simulink model "IFOC_BLOCKS"  (R2025a)
settings: Solver=ode4  StartTime=0.0  StopTime=t_stop  FixedStep=h_step  RelTol=1e-3
InitFcn:
  | addpath(fileparts(get_param('IFOC_BLOCKS','FileName'))); bm_drive = 'IFOC'; bm_model = 'IFOC_BLOCKS'; block_model_params;
values from neighbouring files (symbols this model uses):
  Bm = m.B    [block_model_params.m]
  Esw = P.inv.Esw    [block_model_params.m]
  flux_mode_default = c.flux_mode    [block_model_params.m]
  h_step = 5e-6    (= 5e-06)    [block_model_params.m]
  Iref_sw = P.inv.Iref    [block_model_params.m]
  Jm = m.J    [block_model_params.m]
  ke = m.ke    [block_model_params.m]
  kh = m.kh    [block_model_params.m]
  Ki_i = c.Ki_i    [block_model_params.m]
  Ko = c.Ko    [block_model_params.m]
  Kp_i = c.Kp_i    [block_model_params.m]
  Kp_w = c.Kp_w    [block_model_params.m]
  Llr = m.Llr    [block_model_params.m]
  Lls = m.Lls    [block_model_params.m]
  Lm0 = m.Lm0    [block_model_params.m]
  Lm_rated = m.Lm_rated    [block_model_params.m]
  lut_an = P.lut.psi    [block_model_params.m]
  lut_ml = bm_P.lut.psi; end    [block_model_params.m]
  lut_T = P.lut.T(:)'    [block_model_params.m]
  lut_w = P.lut.w(:)'    [block_model_params.m]
  mlp_b1 = double(bm_M.b1(:))    [block_model_params.m]
  mlp_b2 = double(bm_M.b2)    [block_model_params.m]
  mlp_W1 = double(bm_M.W1)    [block_model_params.m]
  mlp_W2 = double(bm_M.W2(:)')    [block_model_params.m]
  mlp_x_mu = double(bm_M.x_mu(:))    [block_model_params.m]
  mlp_x_sd = double(bm_M.x_sd(:))    [block_model_params.m]
  mlp_y_mu = double(bm_M.y_mu)    [block_model_params.m]
  mlp_y_sd = double(bm_M.y_sd)    [block_model_params.m]
  mras_Ki = c.mras_Ki    [block_model_params.m]
  mras_Kp = c.mras_Kp    [block_model_params.m]
  mras_wc = c.mras_wc    [block_model_params.m]
  NT = round(Ts/h)    [block_log_to_thesis.m]    (also in block_model_params.m = round(Ts/h_step))
  pp = m.p    [block_model_params.m]
  psi_k = m.psi_k    [block_model_params.m]
  rad2rpm = 60/(2*pi)    (= 9.54929658551)    [block_model_params.m]
  rce = P.inv.rce    [block_model_params.m]
  rpm2rad = 2*pi/60    (= 0.10471975512)    [block_model_params.m]
  Rr = m.Rr    [block_model_params.m]
  Rs = m.Rs    [block_model_params.m]
  s32 = sqrt(3)/2    [block_model_params.m]
  sat_a = m.sat_a    [block_model_params.m]
  sat_b = m.sat_b    [block_model_params.m]
  sat_on = m.sat_on    [block_model_params.m]
  speed_mode_default = c.speed_mode    [block_model_params.m]
  t_fault = 0.8    [block_model_params.m]
  Te_max = c.Te_max    [block_model_params.m]
  Ts = P.ctrl.Ts    [block_log_to_thesis.m]    (also in block_model_params.m = c.Ts)
  twopi = 2*pi    (= 6.28318530718)    [block_model_params.m]
  Vce0 = P.inv.Vce0    [block_model_params.m]
  Vdc = P.inv.Vdc    [block_model_params.m]
  Vref_sw = P.inv.Vref    [block_model_params.m]
(part 1 of 2)
settings Model: Creator=ironman  LastModifiedBy=ironman
settings DataIOCC: SaveOutput=off  SignalLogging=off  SaveTime=off

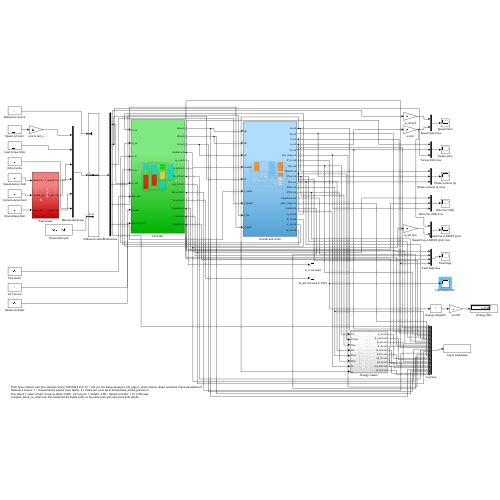
[thumbnail: Simulink's stored preview of the top-level diagram]
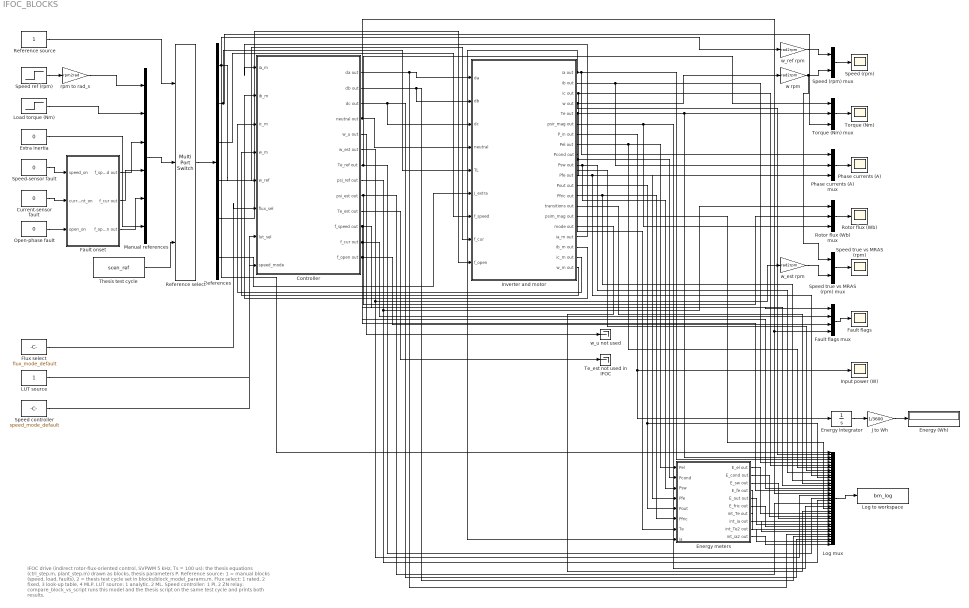
== system IFOC_BLOCKS ==
  note: IFOC drive (indirect rotor-flux-oriented control, SVPWM 5 kHz, Ts = 100 us): the thesis equations (ctrl_step.m, plant_step.m) drawn as blocks, thesis parameters P.
      | Reference source: 1 = manual blocks (speed, load, faults), 2 = thesis test cycle set in blocks/block_model_params.m.
      | Flux select: 1 rated, 2 fixed, 3 look-up table, 4 MLP.  LUT source: 1 analytic, 2 ML.  Speed controller: 1 PI, 2 ZN relay.
      | compare_block_vs_script runs this model and the thesis script on the same test cycle and prints both results.
  Controller : Subsystem
  Current-sensor fault : Constant  Value=0
  Energy (Wh) : Display
  Energy integrator : Integrator
  Energy meters : Subsystem
  Extra inertia : Constant  Value=0
  Fault flags : Scope
      settings: ActiveDisplayYMinimum=-1  ActiveDisplayYMaximum=1
  Fault flags mux : Mux
  Fault onset : Subsystem
  Flux select : Constant  Value=flux_mode_default
  Input power (W) : Scope
      settings: ActiveDisplayYMinimum=-1  ActiveDisplayYMaximum=1
  Inverter and motor : Subsystem
  J to Wh : Gain  Gain=1/3600
  LUT source : Constant
  Load torque (Nm) : Step  Time=0.6  After=13  SampleTime=0
  Log mux : Mux  Inputs=37
  Log to workspace : ToWorkspace  VariableName=bm_log  SaveFormat=Structure With Time  SampleTime=-1
  Manual references : Mux  Inputs=6
  Open-phase fault : Constant  Value=0
  Phase currents (A) : Scope
      settings: ActiveDisplayYMinimum=-1  ActiveDisplayYMaximum=1
  Phase currents (A) mux : Mux  Inputs=3
  Reference select : MultiPortSwitch  Inputs=2  SaturateOnIntegerOverflow=off  InputSameDT=off
  Reference source : Constant
  References : Demux  Outputs=6
  Rotor flux (Wb) : Scope
      settings: ActiveDisplayYMinimum=-1  ActiveDisplayYMaximum=1
  Rotor flux (Wb) mux : Mux  Inputs=3
  Speed (rpm) : Scope
      settings: ActiveDisplayYMinimum=-1  ActiveDisplayYMaximum=1
  Speed (rpm) mux : Mux  Inputs=2
  Speed controller : Constant  Value=speed_mode_default
  Speed ref (rpm) : Step  Time=0.2  After=1000  SampleTime=0
  Speed true vs MRAS (rpm) : Scope
      settings: ActiveDisplayYMinimum=-1  ActiveDisplayYMaximum=1
  Speed true vs MRAS (rpm) mux : Mux  Inputs=2
  Speed-sensor fault : Constant  Value=0
  Te_est not used in IFOC : Terminator
  Thesis test cycle : FromWorkspace  VariableName=scen_ref  SampleTime=Ts  Interpolate=off  OutputAfterFinalValue=Holding final value
  Torque (Nm) : Scope
      settings: ActiveDisplayYMinimum=-1  ActiveDisplayYMaximum=1
  Torque (Nm) mux : Mux  Inputs=3
  rpm to rad_s : Gain  Gain=rpm2rad
  w rpm : Gain  Gain=rad2rpm
  w_est rpm : Gain  Gain=rad2rpm
  w_ref rpm : Gain  Gain=rad2rpm
  w_u not used : Terminator
  wires:
  Speed ref (rpm)/1 -> rpm to rad_s/1
  Speed-sensor fault/1 -> Fault onset/1(speed_on)
  Current-sensor fault/1 -> Fault onset/2(current_on)
  Open-phase fault/1 -> Fault onset/3(open_on)
  rpm to rad_s/1 -> Manual references/1
  Load torque (Nm)/1 -> Manual references/2
  Fault onset/1(f_speed out) -> Manual references/3
  Fault onset/2(f_cur out) -> Manual references/4
  Fault onset/3(f_open out) -> Manual references/5
  Extra inertia/1 -> Manual references/6
  Reference source/1 -> Reference select/1
  Manual references/1 -> Reference select/2
  Thesis test cycle/1 -> Reference select/3
  Reference select/1 -> References/1
  Inverter and motor/17(ia_m out) -> Controller/1(ia_m)
  Inverter and motor/18(ib_m out) -> Controller/2(ib_m)
  Inverter and motor/19(ic_m out) -> Controller/3(ic_m)
  Inverter and motor/20(w_m out) -> Controller/4(w_m)
  References/1 -> Controller/5(w_ref), w_ref rpm/1, Log mux/1
  Flux select/1 -> Controller/6(flux_sel)
  LUT source/1 -> Controller/7(lut_sel)
  Speed controller/1 -> Controller/8(speed_mode)
  Controller/1(da out) -> Inverter and motor/1(da), Log mux/33
  Controller/2(db out) -> Inverter and motor/2(db), Log mux/34
  Controller/3(dc out) -> Inverter and motor/3(dc), Log mux/35
  Controller/4(neutral out) -> Fault flags mux/4, Log mux/17, Inverter and motor/4(neutral)
  References/2 -> Inverter and motor/5(TL), Torque (Nm) mux/3
  References/6 -> Inverter and motor/6(J_extra)
  References/3 -> Inverter and motor/7(f_speed)
  References/4 -> Inverter and motor/8(f_cur)
  References/5 -> Inverter and motor/9(f_open)
  Controller/5(w_u out) -> w_u not used/1
  Controller/10(Te_est out) -> Te_est not used in IFOC/1
  Inverter and motor/4(w out) -> w rpm/1, Log mux/2
  w_ref rpm/1 -> Speed (rpm) mux/1
  w rpm/1 -> Speed (rpm) mux/2, Speed true vs MRAS (rpm) mux/1
  Speed (rpm) mux/1 -> Speed (rpm)/1
  Controller/7(Te_ref out) -> Torque (Nm) mux/1, Log mux/19
  Inverter and motor/5(Te out) -> Torque (Nm) mux/2, Log mux/3, Energy meters/7(Te)
  Torque (Nm) mux/1 -> Torque (Nm)/1
  Controller/8(psi_ref out) -> Rotor flux (Wb) mux/1, Log mux/20
  Controller/9(psi_est out) -> Rotor flux (Wb) mux/2, Log mux/21
  Inverter and motor/6(psir_mag out) -> Rotor flux (Wb) mux/3, Log mux/22
  Rotor flux (Wb) mux/1 -> Rotor flux (Wb)/1
  Inverter and motor/1(ia out) -> Phase currents (A) mux/1, Log mux/4, Energy meters/8(ia)
  Inverter and motor/2(ib out) -> Phase currents (A) mux/2, Log mux/5
  Inverter and motor/3(ic out) -> Phase currents (A) mux/3, Log mux/6
  Phase currents (A) mux/1 -> Phase currents (A)/1
  Controller/6(w_est out) -> w_est rpm/1, Log mux/18
  w_est rpm/1 -> Speed true vs MRAS (rpm) mux/2
  Speed true vs MRAS (rpm) mux/1 -> Speed true vs MRAS (rpm)/1
  Controller/11(f_speed out) -> Fault flags mux/1, Log mux/14
  Controller/12(f_cur out) -> Fault flags mux/2, Log mux/15
  Controller/13(f_open out) -> Fault flags mux/3, Log mux/16
  Fault flags mux/1 -> Fault flags/1
  Inverter and motor/7(P_in out) -> Input power (W)/1, Energy integrator/1
  Energy integrator/1 -> J to Wh/1
  J to Wh/1 -> Energy (Wh)/1
  Inverter and motor/8(Pel out) -> Energy meters/1(Pel), Log mux/7
  Inverter and motor/9(Pcond out) -> Energy meters/2(Pcond), Log mux/8
  Inverter and motor/10(Psw out) -> Energy meters/3(Psw), Log mux/9
  Inverter and motor/11(Pfe out) -> Energy meters/4(Pfe), Log mux/10
  Inverter and motor/12(Pout out) -> Energy meters/5(Pout), Log mux/11
  Inverter and motor/13(Pfric out) -> Energy meters/6(Pfric), Log mux/12
  Inverter and motor/14(transitions out) -> Log mux/13
  Inverter and motor/15(psim_mag out) -> Log mux/23
  Inverter and motor/16(mode out) -> Log mux/24
  Energy meters/1(E_el out) -> Log mux/25
  Energy meters/2(E_cond out) -> Log mux/26
  Energy meters/3(E_sw out) -> Log mux/27
  Energy meters/4(E_fe out) -> Log mux/28
  Energy meters/5(E_out out) -> Log mux/29
  Energy meters/6(E_fric out) -> Log mux/30
  Energy meters/7(int_Te out) -> Log mux/31
  Energy meters/8(int_ia out) -> Log mux/32
  Energy meters/9(int_Te2 out) -> Log mux/36
  Energy meters/10(int_ia2 out) -> Log mux/37
  Log mux/1 -> Log to workspace/1

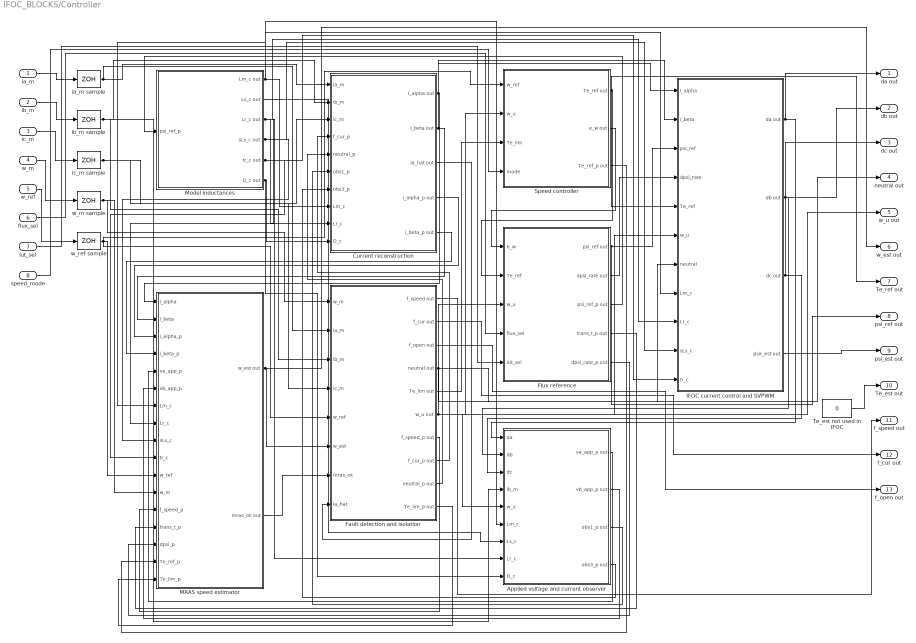
== system IFOC_BLOCKS/Controller ==
  ia_m : Inport
  ib_m : Inport  Port=2
  ic_m : Inport  Port=3
  w_m : Inport  Port=4
  w_ref : Inport  Port=5
  flux_sel : Inport  Port=6
  lut_sel : Inport  Port=7
  speed_mode : Inport  Port=8
  Applied voltage and current observer : Subsystem
  Current reconstruction : Subsystem
  Fault detection and isolation : Subsystem
  Flux reference : Subsystem
  IFOC current control and SVPWM : Subsystem
  MRAS speed estimator : Subsystem
  Model inductances : Subsystem
  Speed controller : Subsystem
  Te_est not used in IFOC : Constant  Value=0
  ia_m sample : ZeroOrderHold  SampleTime=Ts
  ib_m sample : ZeroOrderHold  SampleTime=Ts
  ic_m sample : ZeroOrderHold  SampleTime=Ts
  w_m sample : ZeroOrderHold  SampleTime=Ts
  w_ref sample : ZeroOrderHold  SampleTime=Ts
  da out : Outport
  db out : Outport  Port=2
  dc out : Outport  Port=3
  neutral out : Outport  Port=4
  w_u out : Outport  Port=5
  w_est out : Outport  Port=6
  Te_ref out : Outport  Port=7
  psi_ref out : Outport  Port=8
  psi_est out : Outport  Port=9
  Te_est out : Outport  Port=10
  f_speed out : Outport  Port=11
  f_cur out : Outport  Port=12
  f_open out : Outport  Port=13
  wires:
  ia_m/1 -> ia_m sample/1
  ib_m/1 -> ib_m sample/1
  ic_m/1 -> ic_m sample/1
  w_m/1 -> w_m sample/1
  w_ref/1 -> w_ref sample/1
  Flux reference/3(psi_ref_p out) -> Model inductances/1(psi_ref_p)
  ia_m sample/1 -> Current reconstruction/1(ia_m), Fault detection and isolation/2(ia_m)
  ib_m sample/1 -> Current reconstruction/2(ib_m), Fault detection and isolation/3(ib_m), Applied voltage and current observer/4(ib_m)
  ic_m sample/1 -> Current reconstruction/3(ic_m), Fault detection and isolation/4(ic_m)
  Fault detection and isolation/8(f_cur_p out) -> Current reconstruction/4(f_cur_p)
  Fault detection and isolation/9(neutral_p out) -> Current reconstruction/5(neutral_p)
  Applied voltage and current observer/3(obs1_p out) -> Current reconstruction/6(obs1_p)
  Applied voltage and current observer/4(obs3_p out) -> Current reconstruction/7(obs3_p)
  Model inductances/1(Lm_c out) -> Current reconstruction/8(Lm_c), MRAS speed estimator/7(Lm_c), IFOC current control and SVPWM/8(Lm_c), Applied voltage and current observer/6(Lm_c)
  Model inductances/3(Lr_c out) -> Current reconstruction/9(Lr_c), MRAS speed estimator/8(Lr_c), IFOC current control and SVPWM/9(Lr_c), Applied voltage and current observer/8(Lr_c)
  Model inductances/6(D_c out) -> Current reconstruction/10(D_c), Applied voltage and current observer/9(D_c)
  Current reconstruction/1(i_alpha out) -> MRAS speed estimator/1(i_alpha), IFOC current control and SVPWM/1(i_alpha)
  Current reconstruction/2(i_beta out) -> MRAS speed estimator/2(i_beta), IFOC current control and SVPWM/2(i_beta)
  Current reconstruction/4(i_alpha_p out) -> MRAS speed estimator/3(i_alpha_p)
  Current reconstruction/5(i_beta_p out) -> MRAS speed estimator/4(i_beta_p)
  Applied voltage and current observer/1(va_app_p out) -> MRAS speed estimator/5(va_app_p)
  Applied voltage and current observer/2(vb_app_p out) -> MRAS speed estimator/6(vb_app_p)
  Model inductances/4(sLs_c out) -> MRAS speed estimator/9(sLs_c), IFOC current control and SVPWM/10(sLs_c)
  Model inductances/5(tr_c out) -> MRAS speed estimator/10(tr_c), IFOC current control and SVPWM/11(tr_c)
  w_ref sample/1 -> MRAS speed estimator/11(w_ref), Fault detection and isolation/5(w_ref), Speed controller/1(w_ref)
  w_m sample/1 -> MRAS speed estimator/12(w_m), Fault detection and isolation/1(w_m)
  Fault detection and isolation/7(f_speed_p out) -> MRAS speed estimator/13(f_speed_p)
  Flux reference/4(trans_t_p out) -> MRAS speed estimator/14(trans_t_p)
  Flux reference/5(dpsi_rate_p out) -> MRAS speed estimator/15(dpsi_p)
  Speed controller/3(Te_ref_p out) -> MRAS speed estimator/16(Te_ref_p)
  Fault detection and isolation/10(Te_lim_p out) -> MRAS speed estimator/17(Te_lim_p)
  MRAS speed estimator/1(w_est out) -> Fault detection and isolation/6(w_est), w_est out/1
  MRAS speed estimator/2(mras_ok out) -> Fault detection and isolation/7(mras_ok)
  Current reconstruction/3(ia_hat out) -> Fault detection and isolation/8(ia_hat)
  Fault detection and isolation/6(w_u out) -> Speed controller/2(w_u), Flux reference/3(w_u), IFOC current control and SVPWM/6(w_u), Applied voltage and current observer/5(w_u), w_u out/1
  Fault detection and isolation/5(Te_lim out) -> Speed controller/3(Te_lim)
  speed_mode/1 -> Speed controller/4(mode)
  Speed controller/2(e_w out) -> Flux reference/1(e_w)
  Speed controller/1(Te_ref out) -> Flux reference/2(Te_ref), IFOC current control and SVPWM/5(Te_ref), Te_ref out/1
  flux_sel/1 -> Flux reference/4(flux_sel)
  lut_sel/1 -> Flux reference/5(lut_sel)
  Flux reference/1(psi_ref out) -> IFOC current control and SVPWM/3(psi_ref), psi_ref out/1
  Flux reference/2(dpsi_rate out) -> IFOC current control and SVPWM/4(dpsi_rate)
  Fault detection and isolation/4(neutral out) -> IFOC current control and SVPWM/7(neutral), neutral out/1
  Te_est not used in IFOC/1 -> Te_est out/1
  IFOC current control and SVPWM/1(da out) -> Applied voltage and current observer/1(da), da out/1
  IFOC current control and SVPWM/2(db out) -> Applied voltage and current observer/2(db), db out/1
  IFOC current control and SVPWM/3(dc out) -> Applied voltage and current observer/3(dc), dc out/1
  Model inductances/2(Ls_c out) -> Applied voltage and current observer/7(Ls_c)
  IFOC current control and SVPWM/4(psir_est out) -> psi_est out/1
  Fault detection and isolation/1(f_speed out) -> f_speed out/1
  Fault detection and isolation/2(f_cur out) -> f_cur out/1
  Fault detection and isolation/3(f_open out) -> f_open out/1

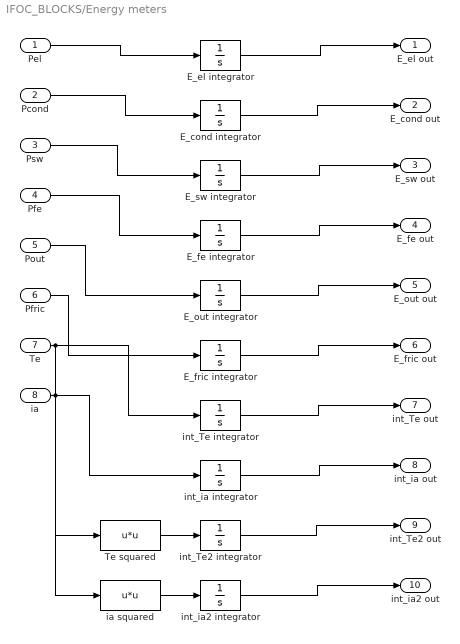
== system IFOC_BLOCKS/Energy meters ==
  Pel : Inport
  Pcond : Inport  Port=2
  Psw : Inport  Port=3
  Pfe : Inport  Port=4
  Pout : Inport  Port=5
  Pfric : Inport  Port=6
  Te : Inport  Port=7
  ia : Inport  Port=8
  E_cond integrator : Integrator
  E_el integrator : Integrator
  E_fe integrator : Integrator
  E_fric integrator : Integrator
  E_out integrator : Integrator
  E_sw integrator : Integrator
  Te squared : Fcn  Expr=u*u
  ia squared : Fcn  Expr=u*u
  int_Te integrator : Integrator
  int_Te2 integrator : Integrator
  int_ia integrator : Integrator
  int_ia2 integrator : Integrator
  E_el out : Outport
  E_cond out : Outport  Port=2
  E_sw out : Outport  Port=3
  E_fe out : Outport  Port=4
  E_out out : Outport  Port=5
  E_fric out : Outport  Port=6
  int_Te out : Outport  Port=7
  int_ia out : Outport  Port=8
  int_Te2 out : Outport  Port=9
  int_ia2 out : Outport  Port=10
  wires:
  Pel/1 -> E_el integrator/1
  E_el integrator/1 -> E_el out/1
  Pcond/1 -> E_cond integrator/1
  E_cond integrator/1 -> E_cond out/1
  Psw/1 -> E_sw integrator/1
  E_sw integrator/1 -> E_sw out/1
  Pfe/1 -> E_fe integrator/1
  E_fe integrator/1 -> E_fe out/1
  Pout/1 -> E_out integrator/1
  E_out integrator/1 -> E_out out/1
  Pfric/1 -> E_fric integrator/1
  E_fric integrator/1 -> E_fric out/1
  Te/1 -> int_Te integrator/1, Te squared/1
  int_Te integrator/1 -> int_Te out/1
  ia/1 -> int_ia integrator/1, ia squared/1
  int_ia integrator/1 -> int_ia out/1
  Te squared/1 -> int_Te2 integrator/1
  int_Te2 integrator/1 -> int_Te2 out/1
  ia squared/1 -> int_ia2 integrator/1
  int_ia2 integrator/1 -> int_ia2 out/1

== system IFOC_BLOCKS/Fault onset ==
  speed_on : Inport
  current_on : Inport  Port=2
  open_on : Inport  Port=3
  Active 1 : Product
  Active 2 : Product
  Active 3 : Product
  Fault time : Step  Time=t_fault  SampleTime=0
  f_speed out : Outport
  f_cur out : Outport  Port=2
  f_open out : Outport  Port=3
  wires:
  speed_on/1 -> Active 1/1
  Fault time/1 -> Active 1/2, Active 2/2, Active 3/2
  Active 1/1 -> f_speed out/1
  current_on/1 -> Active 2/1
  Active 2/1 -> f_cur out/1
  open_on/1 -> Active 3/1
  Active 3/1 -> f_open out/1

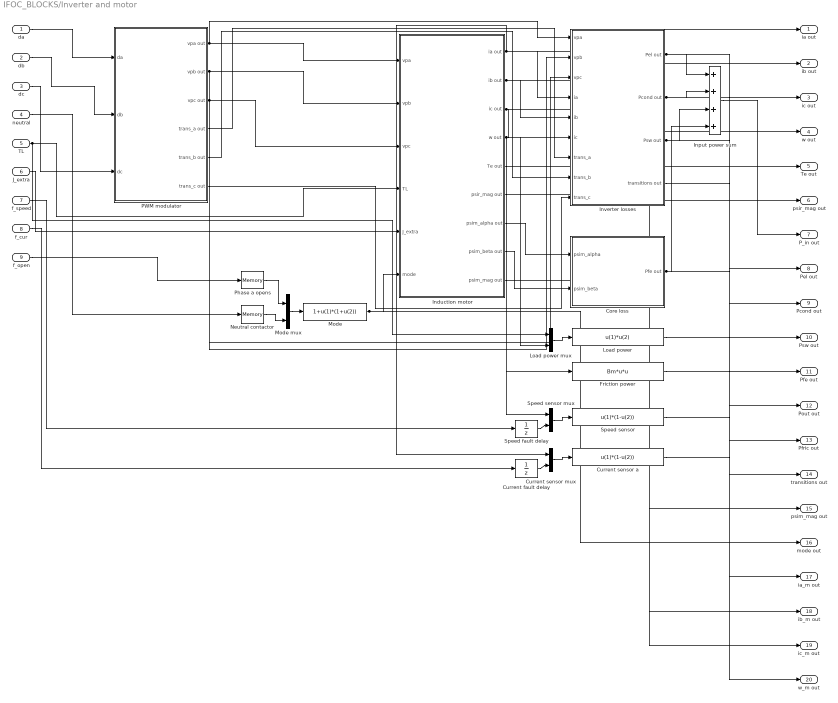
== system IFOC_BLOCKS/Inverter and motor ==
  da : Inport
  db : Inport  Port=2
  dc : Inport  Port=3
  neutral : Inport  Port=4
  TL : Inport  Port=5
  J_extra : Inport  Port=6
  f_speed : Inport  Port=7
  f_cur : Inport  Port=8
  f_open : Inport  Port=9
  Core loss : Subsystem
  Current fault delay : UnitDelay  SampleTime=Ts  HasFrameUpgradeWarning=on
  Current sensor a : Fcn  Expr=u(1)*(1-u(2))
  Current sensor mux : Mux  Inputs=2
  Friction power : Fcn  Expr=Bm*u*u
  Induction motor : Subsystem
  Input power sum : Sum  Inputs=++++
  Inverter losses : Subsystem
  Load power : Fcn  Expr=u(1)*u(2)
  Load power mux : Mux  Inputs=2
  Mode : Fcn  Expr=1+u(1)*(1+u(2))
  Mode mux : Mux  Inputs=2
  Neutral contactor : Memory
  PWM modulator : Subsystem
  Phase a opens : Memory
  Speed fault delay : UnitDelay  SampleTime=Ts  HasFrameUpgradeWarning=on
  Speed sensor : Fcn  Expr=u(1)*(1-u(2))
  Speed sensor mux : Mux  Inputs=2
  ia out : Outport
  ib out : Outport  Port=2
  ic out : Outport  Port=3
  w out : Outport  Port=4
  Te out : Outport  Port=5
  psir_mag out : Outport  Port=6
  P_in out : Outport  Port=7
  Pel out : Outport  Port=8
  Pcond out : Outport  Port=9
  Psw out : Outport  Port=10
  Pfe out : Outport  Port=11
  Pout out : Outport  Port=12
  Pfric out : Outport  Port=13
  transitions out : Outport  Port=14
  psim_mag out : Outport  Port=15
  mode out : Outport  Port=16
  ia_m out : Outport  Port=17
  ib_m out : Outport  Port=18
  ic_m out : Outport  Port=19
  w_m out : Outport  Port=20
  wires:
  neutral/1 -> Neutral contactor/1
  f_open/1 -> Phase a opens/1
  Phase a opens/1 -> Mode mux/1
  Neutral contactor/1 -> Mode mux/2
  Mode mux/1 -> Mode/1
  da/1 -> PWM modulator/1(da)
  db/1 -> PWM modulator/2(db)
  dc/1 -> PWM modulator/3(dc)
  PWM modulator/1(vpa out) -> Induction motor/1(vpa), Inverter losses/1(vpa)
  PWM modulator/2(vpb out) -> Induction motor/2(vpb), Inverter losses/2(vpb)
  PWM modulator/3(vpc out) -> Induction motor/3(vpc), Inverter losses/3(vpc)
  TL/1 -> Induction motor/4(TL), Load power mux/1
  J_extra/1 -> Induction motor/5(J_extra)
  Mode/1 -> Induction motor/6(mode), mode out/1
  Induction motor/1(ia out) -> Inverter losses/4(ia), Current sensor mux/1, ia out/1
  PWM modulator/4(trans_a out) -> Inverter losses/7(trans_a)
  Induction motor/2(ib out) -> Inverter losses/5(ib), ib out/1, ib_m out/1
  PWM modulator/5(trans_b out) -> Inverter losses/8(trans_b)
  Induction motor/3(ic out) -> Inverter losses/6(ic), ic out/1, ic_m out/1
  PWM modulator/6(trans_c out) -> Inverter losses/9(trans_c)
  Induction motor/7(psim_alpha out) -> Core loss/1(psim_alpha)
  Induction motor/8(psim_beta out) -> Core loss/2(psim_beta)
  Induction motor/4(w out) -> Load power mux/2, Friction power/1, Speed sensor mux/1, w out/1
  Load power mux/1 -> Load power/1
  Inverter losses/1(Pel out) -> Input power sum/1, Pel out/1
  Inverter losses/2(Pcond out) -> Input power sum/2, Pcond out/1
  Inverter losses/3(Psw out) -> Input power sum/3, Psw out/1
  Core loss/1(Pfe out) -> Input power sum/4, Pfe out/1
  f_speed/1 -> Speed fault delay/1
  f_cur/1 -> Current fault delay/1
  Speed fault delay/1 -> Speed sensor mux/2
  Speed sensor mux/1 -> Speed sensor/1
  Current fault delay/1 -> Current sensor mux/2
  Current sensor mux/1 -> Current sensor a/1
  Induction motor/5(Te out) -> Te out/1
  Induction motor/6(psir_mag out) -> psir_mag out/1
  Input power sum/1 -> P_in out/1
  Load power/1 -> Pout out/1
  Friction power/1 -> Pfric out/1
  Inverter losses/4(transitions out) -> transitions out/1
  Induction motor/9(psim_mag out) -> psim_mag out/1
  Current sensor a/1 -> ia_m out/1
  Speed sensor/1 -> w_m out/1

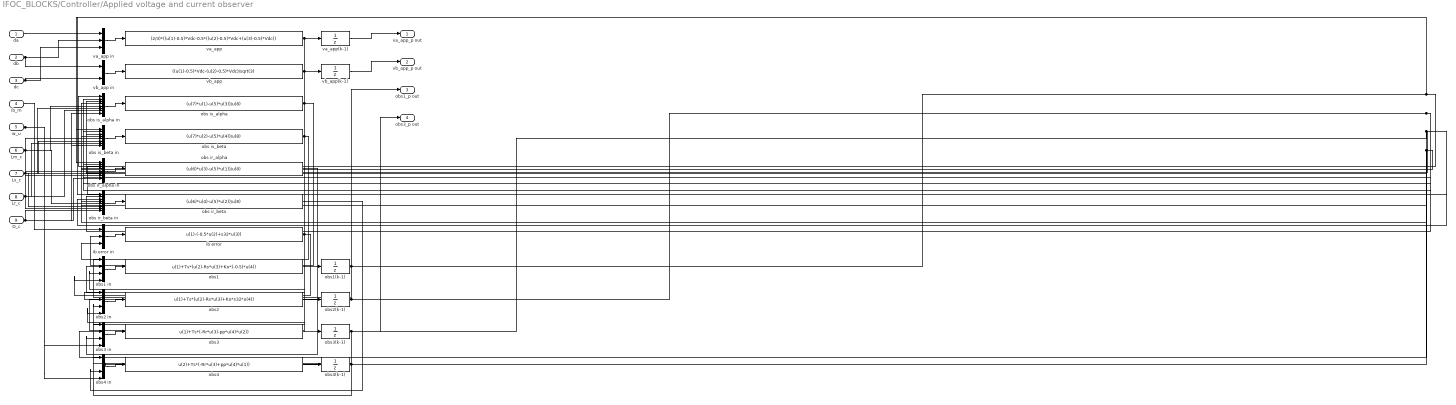
== system IFOC_BLOCKS/Controller/Applied voltage and current observer ==
  da : Inport
  db : Inport  Port=2
  dc : Inport  Port=3
  ib_m : Inport  Port=4
  w_u : Inport  Port=5
  Lm_c : Inport  Port=6
  Ls_c : Inport  Port=7
  Lr_c : Inport  Port=8
  D_c : Inport  Port=9
  ib error : Fcn  Expr=u(1)-(-0.5*u(2)+s32*u(3))
  ib error in : Mux  Inputs=3
  obs ir_alpha : Fcn  Expr=(u(6)*u(3)-u(5)*u(1))/u(8)
  obs ir_alpha in : Mux  Inputs=8
  obs ir_beta : Fcn  Expr=(u(6)*u(4)-u(5)*u(2))/u(8)
  obs ir_beta in : Mux  Inputs=8
  obs is_alpha : Fcn  Expr=(u(7)*u(1)-u(5)*u(3))/u(8)
  obs is_alpha in : Mux  Inputs=8
  obs is_beta : Fcn  Expr=(u(7)*u(2)-u(5)*u(4))/u(8)
  obs is_beta in : Mux  Inputs=8
  obs1 : Fcn  Expr=u(1)+Ts*(u(2)-Rs*u(3)+Ko*(-0.5)*u(4))
  obs1 in : Mux
  obs1(k-1) : UnitDelay  SampleTime=Ts  HasFrameUpgradeWarning=on
  obs2 : Fcn  Expr=u(1)+Ts*(u(2)-Rs*u(3)+Ko*s32*u(4))
  obs2 in : Mux
  obs2(k-1) : UnitDelay  SampleTime=Ts  HasFrameUpgradeWarning=on
  obs3 : Fcn  Expr=u(1)+Ts*(-Rr*u(3)-pp*u(4)*u(2))
  obs3 in : Mux
  obs3(k-1) : UnitDelay  SampleTime=Ts  HasFrameUpgradeWarning=on
  obs4 : Fcn  Expr=u(2)+Ts*(-Rr*u(3)+pp*u(4)*u(1))
  obs4 in : Mux
  obs4(k-1) : UnitDelay  SampleTime=Ts  HasFrameUpgradeWarning=on
  va_app : Fcn  Expr=(2/3)*((u(1)-0.5)*Vdc-0.5*((u(2)-0.5)*Vdc+(u(3)-0.5)*Vdc))
  va_app in : Mux  Inputs=3
  va_app(k-1) : UnitDelay  SampleTime=Ts  HasFrameUpgradeWarning=on
  vb_app : Fcn  Expr=((u(1)-0.5)*Vdc-(u(2)-0.5)*Vdc)/sqrt(3)
  vb_app in : Mux  Inputs=2
  vb_app(k-1) : UnitDelay  SampleTime=Ts  HasFrameUpgradeWarning=on
  va_app_p out : Outport
  vb_app_p out : Outport  Port=2
  obs1_p out : Outport  Port=3
  obs3_p out : Outport  Port=4
  wires:
  da/1 -> va_app in/1
  db/1 -> va_app in/2, vb_app in/1
  dc/1 -> va_app in/3, vb_app in/2
  va_app in/1 -> va_app/1
  va_app/1 -> va_app(k-1)/1, obs1 in/2
  vb_app in/1 -> vb_app/1
  vb_app/1 -> vb_app(k-1)/1, obs2 in/2
  obs1(k-1)/1 -> obs is_alpha in/1, obs is_beta in/1, obs ir_alpha in/1, obs ir_beta in/1, obs1 in/1, obs1_p out/1
  obs2(k-1)/1 -> obs is_alpha in/2, obs is_beta in/2, obs ir_alpha in/2, obs ir_beta in/2, obs2 in/1
  obs3(k-1)/1 -> obs is_alpha in/3, obs is_beta in/3, obs ir_alpha in/3, obs ir_beta in/3, obs3 in/1, obs4 in/1, obs3_p out/1
  obs4(k-1)/1 -> obs is_alpha in/4, obs is_beta in/4, obs ir_alpha in/4, obs ir_beta in/4, obs3 in/2, obs4 in/2
  Lm_c/1 -> obs is_alpha in/5, obs is_beta in/5, obs ir_alpha in/5, obs ir_beta in/5
  Ls_c/1 -> obs is_alpha in/6, obs is_beta in/6, obs ir_alpha in/6, obs ir_beta in/6
  Lr_c/1 -> obs is_alpha in/7, obs is_beta in/7, obs ir_alpha in/7, obs ir_beta in/7
  D_c/1 -> obs is_alpha in/8, obs is_beta in/8, obs ir_alpha in/8, obs ir_beta in/8
  obs is_alpha in/1 -> obs is_alpha/1
  obs is_beta in/1 -> obs is_beta/1
  obs ir_alpha in/1 -> obs ir_alpha/1
  obs ir_beta in/1 -> obs ir_beta/1
  ib_m/1 -> ib error in/1
  obs is_alpha/1 -> ib error in/2, obs1 in/3
  obs is_beta/1 -> ib error in/3, obs2 in/3
  ib error in/1 -> ib error/1
  ib error/1 -> obs1 in/4, obs2 in/4
  obs1 in/1 -> obs1/1
  obs1/1 -> obs1(k-1)/1
  obs2 in/1 -> obs2/1
  obs2/1 -> obs2(k-1)/1
  obs ir_alpha/1 -> obs3 in/3
  w_u/1 -> obs3 in/4, obs4 in/4
  obs3 in/1 -> obs3/1
  obs3/1 -> obs3(k-1)/1
  obs ir_beta/1 -> obs4 in/3
  obs4 in/1 -> obs4/1
  obs4/1 -> obs4(k-1)/1
  va_app(k-1)/1 -> va_app_p out/1
  vb_app(k-1)/1 -> vb_app_p out/1

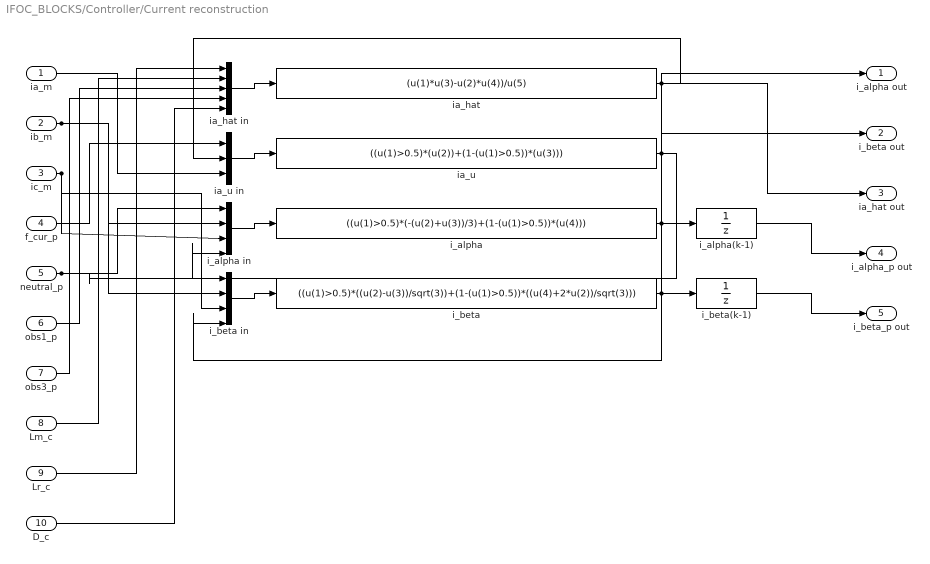
== system IFOC_BLOCKS/Controller/Current reconstruction ==
  ia_m : Inport
  ib_m : Inport  Port=2
  ic_m : Inport  Port=3
  f_cur_p : Inport  Port=4
  neutral_p : Inport  Port=5
  obs1_p : Inport  Port=6
  obs3_p : Inport  Port=7
  Lm_c : Inport  Port=8
  Lr_c : Inport  Port=9
  D_c : Inport  Port=10
  i_alpha : Fcn  Expr=((u(1)>0.5)*(-(u(2)+u(3))/3)+(1-(u(1)>0.5))*(u(4)))
  i_alpha in : Mux
  i_alpha(k-1) : UnitDelay  SampleTime=Ts  HasFrameUpgradeWarning=on
  i_beta : Fcn  Expr=((u(1)>0.5)*((u(2)-u(3))/sqrt(3))+(1-(u(1)>0.5))*((u(4)+2*u(2))/sqrt(3)))
  i_beta in : Mux
  i_beta(k-1) : UnitDelay  SampleTime=Ts  HasFrameUpgradeWarning=on
  ia_hat : Fcn  Expr=(u(1)*u(3)-u(2)*u(4))/u(5)
  ia_hat in : Mux  Inputs=5
  ia_u : Fcn  Expr=((u(1)>0.5)*(u(2))+(1-(u(1)>0.5))*(u(3)))
  ia_u in : Mux  Inputs=3
  i_alpha out : Outport
  i_beta out : Outport  Port=2
  ia_hat out : Outport  Port=3
  i_alpha_p out : Outport  Port=4
  i_beta_p out : Outport  Port=5
  wires:
  Lr_c/1 -> ia_hat in/1
  Lm_c/1 -> ia_hat in/2
  obs1_p/1 -> ia_hat in/3
  obs3_p/1 -> ia_hat in/4
  D_c/1 -> ia_hat in/5
  ia_hat in/1 -> ia_hat/1
  f_cur_p/1 -> ia_u in/1
  ia_hat/1 -> ia_u in/2, ia_hat out/1
  ia_m/1 -> ia_u in/3
  ia_u in/1 -> ia_u/1
  neutral_p/1 -> i_alpha in/1, i_beta in/1
  ib_m/1 -> i_alpha in/2, i_beta in/2
  ic_m/1 -> i_alpha in/3, i_beta in/3
  ia_u/1 -> i_alpha in/4, i_beta in/4
  i_alpha in/1 -> i_alpha/1
  i_alpha/1 -> i_alpha(k-1)/1, i_alpha out/1
  i_beta in/1 -> i_beta/1
  i_beta/1 -> i_beta(k-1)/1, i_beta out/1
  i_alpha(k-1)/1 -> i_alpha_p out/1
  i_beta(k-1)/1 -> i_beta_p out/1

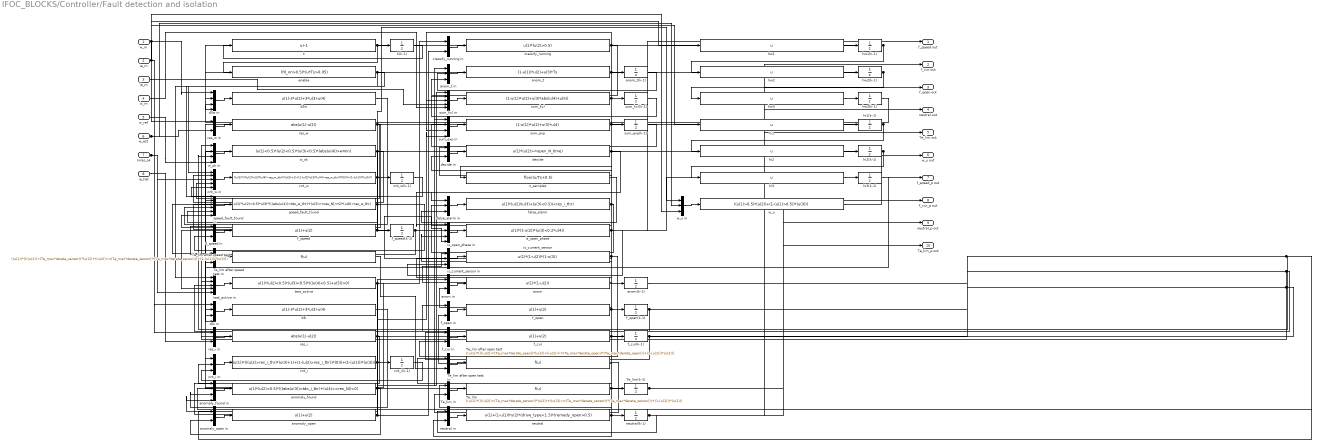
== system IFOC_BLOCKS/Controller/Fault detection and isolation ==
  w_m : Inport
  ia_m : Inport  Port=2
  ib_m : Inport  Port=3
  ic_m : Inport  Port=4
  w_ref : Inport  Port=5
  w_est : Inport  Port=6
  mras_ok : Inport  Port=7
  ia_hat : Inport  Port=8
  Te_lim : Fcn  Expr=((u(1))*((((u(2))<(Te_max*derate_sensor))*(u(2))+((u(2))>=(Te_max*derate_sensor))*(Te_max*derate_sensor)))+(1-(u(1)))*(u(2)))
  Te_lim after open test : Fcn  Expr=((u(1))*((((u(2))<(Te_max*derate_open))*(u(2))+((u(2))>=(Te_max*derate_open))*(Te_max*derate_open)))+(1-(u(1)))*(u(2)))
  Te_lim after open test in : Mux  Inputs=2
  Te_lim after speed test : Fcn  Expr=((u(1))*((((u(2))<(Te_max*derate_sensor))*(u(2))+((u(2))>=(Te_max*derate_sensor))*(Te_max*derate_sensor)))+(1-(u(1)))*(u(2)))
  Te_lim after speed test in : Mux  Inputs=2
  Te_lim in : Mux  Inputs=2
  Te_lim(k-1) : UnitDelay  InitialCondition=Te_max  SampleTime=Ts  HasFrameUpgradeWarning=on
  anom : Fcn  Expr=u(1)*(1-u(2))
  anom in : Mux  Inputs=2
  anom(k-1) : UnitDelay  SampleTime=Ts  HasFrameUpgradeWarning=on
  anom_t : Fcn  Expr=(1-u(1))*u(2)+u(3)*Ts
  anom_t in : Mux  Inputs=3
  anom_t(k-1) : UnitDelay  SampleTime=Ts  HasFrameUpgradeWarning=on
  anomaly_found : Fcn  Expr=u(1)*(u(2)<0.5)*(((abs(u(3))>tdo_i_thr)+(u(4)>=res_N))>0)
  anomaly_found in : Mux
  anomaly_open : Fcn  Expr=u(1)+u(2)
  anomaly_open in : Mux  Inputs=2
  classify_running : Fcn  Expr=u(1)*(u(2)>0.5)
  classify_running in : Mux  Inputs=2
  cnt_i : Fcn  Expr=((u(1))*(((u(2)>res_i_thr)*(u(3)+1)+(1-(u(2)>res_i_thr))*(0)))+(1-(u(1)))*(u(3)))
  cnt_i in : Mux  Inputs=3
  cnt_i(k-1) : UnitDelay  SampleTime=Ts  HasFrameUpgradeWarning=on
  cnt_w : Fcn  Expr=((u(1))*(((u(2)*u(3)*(u(4)>res_w_thr))*(u(5)+1)+(1-(u(2)*u(3)*(u(4)>res_w_thr)))*(0)))+(1-(u(1)))*(u(5)))
  cnt_w in : Mux  Inputs=5
  cnt_w(k-1) : UnitDelay  SampleTime=Ts  HasFrameUpgradeWarning=on
  d3i : Fcn  Expr=u(1)-3*u(2)+3*u(3)-u(4)
  d3i in : Mux
  d3w : Fcn  Expr=u(1)-3*u(2)+3*u(3)-u(4)
  d3w in : Mux
  decide : Fcn  Expr=u(1)*(u(2)>=open_N_time)
  decide in : Mux  Inputs=2
  enable : Fcn  Expr=(fd_on>0.5)*(u*Ts>0.05)
  f_cur : Fcn  Expr=u(1)+u(2)
  f_cur in : Mux  Inputs=2
  f_cur(k-1) : UnitDelay  SampleTime=Ts  HasFrameUpgradeWarning=on
  f_open : Fcn  Expr=u(1)+u(2)
  f_open in : Mux  Inputs=2
  f_open(k-1) : UnitDelay  SampleTime=Ts  HasFrameUpgradeWarning=on
  f_speed : Fcn  Expr=u(1)+u(2)
  f_speed in : Mux  Inputs=2
  f_speed(k-1) : UnitDelay  SampleTime=Ts  HasFrameUpgradeWarning=on
  false_alarm : Fcn  Expr=u(1)*(u(2)/(u(3)+(u(3)<0.5))<res_i_thr)
  false_alarm in : Mux  Inputs=3
  hi1 : Fcn  Expr=u
  hi1(k-1) : UnitDelay  SampleTime=Ts  HasFrameUpgradeWarning=on
  hi2 : Fcn  Expr=u
  hi2(k-1) : UnitDelay  SampleTime=Ts  HasFrameUpgradeWarning=on
  hi3 : Fcn  Expr=u
  hi3(k-1) : UnitDelay  SampleTime=Ts  HasFrameUpgradeWarning=on
  hw1 : Fcn  Expr=u
  hw1(k-1) : UnitDelay  SampleTime=Ts  HasFrameUpgradeWarning=on
  hw2 : Fcn  Expr=u
  hw2(k-1) : UnitDelay  SampleTime=Ts  HasFrameUpgradeWarning=on
  hw3 : Fcn  Expr=u
  hw3(k-1) : UnitDelay  SampleTime=Ts  HasFrameUpgradeWarning=on
  is_current_sensor : Fcn  Expr=u(1)*(1-u(2))*(1-u(3))
  is_current_sensor in : Mux  Inputs=3
  is_open_phase : Fcn  Expr=u(1)*(1-u(2))*(u(3)<0.2*u(4))
  is_open_phase in : Mux
  k : Fcn  Expr=u+1
  k(k-1) : UnitDelay  SampleTime=Ts  HasFrameUpgradeWarning=on
  n_samples : Fcn  Expr=floor(u/Ts+0.5)
  neutral : Fcn  Expr=u(1)+(1-u(1))*u(2)*(drive_type<1.5)*(remedy_open>0.5)
  neutral in : Mux  Inputs=2
  neutral(k-1) : UnitDelay  SampleTime=Ts  HasFrameUpgradeWarning=on
  res_i : Fcn  Expr=abs(u(1)-u(2))
  res_i in : Mux  Inputs=2
  res_w : Fcn  Expr=abs(u(1)-u(2))
  res_w in : Mux  Inputs=2
  speed_fault_found : Fcn  Expr=u(1)*(u(2)<0.5)*u(3)*(((abs(u(4))>tdo_w_thr)+(u(5)>=res_N))>0)*(u(6)>res_w_thr)
  speed_fault_found in : Mux  Inputs=6
  sum_exp : Fcn  Expr=(1-u(1))*u(2)+u(3)*u(4)
  sum_exp in : Mux
  sum_exp(k-1) : UnitDelay  SampleTime=Ts  HasFrameUpgradeWarning=on
  sum_kcl : Fcn  Expr=(1-u(1))*u(2)+u(3)*abs(u(4)+u(5))
  sum_kcl in : Mux  Inputs=5
  sum_kcl(k-1) : UnitDelay  SampleTime=Ts  HasFrameUpgradeWarning=on
  test_active : Fcn  Expr=u(1)*(u(2)<0.5)*(u(3)<0.5)*(((u(4)<0.5)+u(5))>0)
  test_active in : Mux  Inputs=5
  w_ok : Fcn  Expr=(u(1)<0.5)*(u(2)<0.5)*(u(3)<0.5)*(abs(u(4))>wmin)
  w_ok in : Mux
  w_u : Fcn  Expr=((u(1)>0.5)*(u(2))+(1-(u(1)>0.5))*(u(3)))
  w_u in : Mux  Inputs=3
  f_speed out : Outport
  f_cur out : Outport  Port=2
  f_open out : Outport  Port=3
  neutral out : Outport  Port=4
  Te_lim out : Outport  Port=5
  w_u out : Outport  Port=6
  f_speed_p out : Outport  Port=7
  f_cur_p out : Outport  Port=8
  neutral_p out : Outport  Port=9
  Te_lim_p out : Outport  Port=10
  wires:
  k(k-1)/1 -> k/1
  k/1 -> k(k-1)/1, enable/1
  w_m/1 -> d3w in/1, res_w in/1, hw1/1, w_u in/3
  hw1(k-1)/1 -> d3w in/2, hw2/1
  hw2(k-1)/1 -> d3w in/3, hw3/1
  hw3(k-1)/1 -> d3w in/4
  d3w in/1 -> d3w/1
  w_est/1 -> res_w in/2, w_u in/2
  res_w in/1 -> res_w/1
  f_cur(k-1)/1 -> w_ok in/1, test_active in/2, f_cur in/1, f_cur_p out/1
  f_open(k-1)/1 -> w_ok in/2, test_active in/3, f_open in/1
  anom(k-1)/1 -> w_ok in/3, anomaly_found in/2, anomaly_open in/1
  w_ref/1 -> w_ok in/4
  w_ok in/1 -> w_ok/1
  enable/1 -> cnt_w in/1, speed_fault_found in/1, test_active in/1
  w_ok/1 -> cnt_w in/2, speed_fault_found in/3
  mras_ok/1 -> cnt_w in/3, test_active in/5
  res_w/1 -> cnt_w in/4, speed_fault_found in/6
  cnt_w(k-1)/1 -> cnt_w in/5
  cnt_w in/1 -> cnt_w/1
  cnt_w/1 -> cnt_w(k-1)/1, speed_fault_found in/5
  f_speed(k-1)/1 -> speed_fault_found in/2, f_speed in/1, f_speed_p out/1
  d3w/1 -> speed_fault_found in/4
  speed_fault_found in/1 -> speed_fault_found/1
  speed_fault_found/1 -> f_speed in/2, Te_lim after speed test in/1
  f_speed in/1 -> f_speed/1
  f_speed/1 -> f_speed(k-1)/1, test_active in/4, w_u in/1, f_speed out/1
  Te_lim(k-1)/1 -> Te_lim after speed test in/2, Te_lim_p out/1
  Te_lim after speed test in/1 -> Te_lim after speed test/1
  test_active in/1 -> test_active/1
  ia_m/1 -> d3i in/1, res_i in/1, hi1/1
  hi1(k-1)/1 -> d3i in/2, hi2/1
  hi2(k-1)/1 -> d3i in/3, hi3/1
  hi3(k-1)/1 -> d3i in/4
  d3i in/1 -> d3i/1
  ia_hat/1 -> res_i in/2
  res_i in/1 -> res_i/1
  test_active/1 -> cnt_i in/1, anomaly_found in/1, classify_running in/1
  res_i/1 -> cnt_i in/2, sum_exp in/4
  cnt_i(k-1)/1 -> cnt_i in/3
  cnt_i in/1 -> cnt_i/1
  cnt_i/1 -> cnt_i(k-1)/1, anomaly_found in/4
  d3i/1 -> anomaly_found in/3
  anomaly_found in/1 -> anomaly_found/1
  anomaly_found/1 -> anomaly_open in/2, anom_t in/1, sum_kcl in/1, sum_exp in/1
  anomaly_open in/1 -> anomaly_open/1
  anomaly_open/1 -> classify_running in/2, anom in/1
  classify_running in/1 -> classify_running/1
  anom_t(k-1)/1 -> anom_t in/2
  classify_running/1 -> anom_t in/3, sum_kcl in/3, sum_exp in/3, decide in/1
  anom_t in/1 -> anom_t/1
  anom_t/1 -> anom_t(k-1)/1, decide in/2, n_samples/1
  sum_kcl(k-1)/1 -> sum_kcl in/2
  ib_m/1 -> sum_kcl in/4
  ic_m/1 -> sum_kcl in/5
  sum_kcl in/1 -> sum_kcl/1
  sum_kcl/1 -> sum_kcl(k-1)/1, is_open_phase in/3
  sum_exp(k-1)/1 -> sum_exp in/2
  sum_exp in/1 -> sum_exp/1
  sum_exp/1 -> sum_exp(k-1)/1, false_alarm in/2, is_open_phase in/4
  decide in/1 -> decide/1
  decide/1 -> false_alarm in/1, is_open_phase in/1, is_current_sensor in/1, anom in/2
  n_samples/1 -> false_alarm in/3
  false_alarm in/1 -> false_alarm/1
  false_alarm/1 -> is_open_phase in/2, is_current_sensor in/2
  is_open_phase in/1 -> is_open_phase/1
  is_open_phase/1 -> is_current_sensor in/3, f_open in/2, Te_lim after open test in/1, neutral in/2
  is_current_sensor in/1 -> is_current_sensor/1
  anom in/1 -> anom/1
  anom/1 -> anom(k-1)/1
  f_open in/1 -> f_open/1
  f_open/1 -> f_open(k-1)/1, f_open out/1
  is_current_sensor/1 -> f_cur in/2, Te_lim in/1
  f_cur in/1 -> f_cur/1
  f_cur/1 -> f_cur(k-1)/1, f_cur out/1
  Te_lim after speed test/1 -> Te_lim after open test in/2
  Te_lim after open test in/1 -> Te_lim after open test/1
  Te_lim after open test/1 -> Te_lim in/2
  Te_lim in/1 -> Te_lim/1
  Te_lim/1 -> Te_lim(k-1)/1, Te_lim out/1
  neutral(k-1)/1 -> neutral in/1, neutral_p out/1
  neutral in/1 -> neutral/1
  neutral/1 -> neutral(k-1)/1, neutral out/1
  hw1/1 -> hw1(k-1)/1
  hw2/1 -> hw2(k-1)/1
  hw3/1 -> hw3(k-1)/1
  hi1/1 -> hi1(k-1)/1
  hi2/1 -> hi2(k-1)/1
  hi3/1 -> hi3(k-1)/1
  w_u in/1 -> w_u/1
  w_u/1 -> w_u out/1

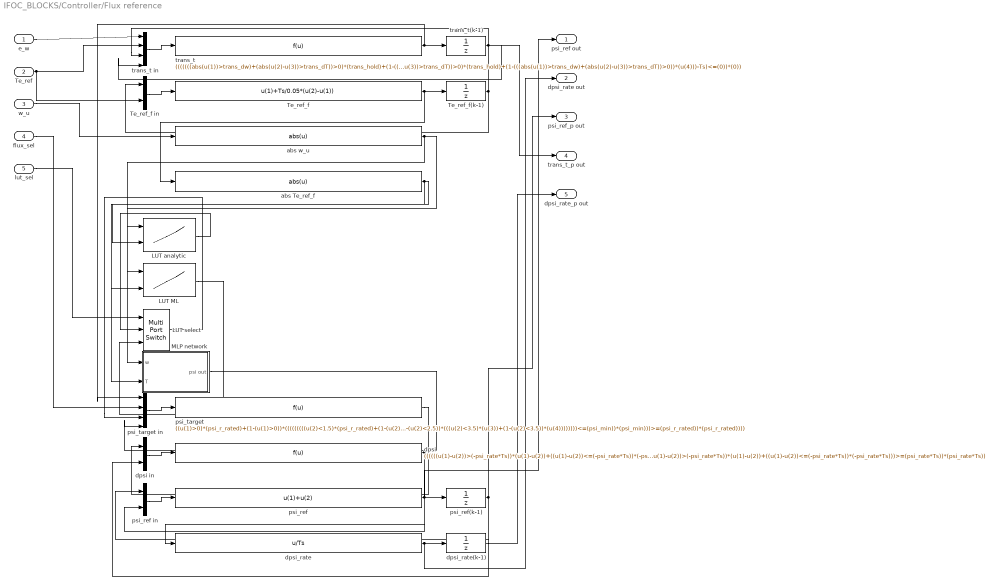
== system IFOC_BLOCKS/Controller/Flux reference ==
  e_w : Inport
  Te_ref : Inport  Port=2
  w_u : Inport  Port=3
  flux_sel : Inport  Port=4
  lut_sel : Inport  Port=5
  LUT ML : Lookup_n-D  BreakpointsForDimension1=lut_w  BreakpointsForDimension2=lut_T  Table=lut_ml  ExtrapMethod=Clip  InternalRulePriority=Speed  RndMeth=Simplest
      settings: InputPortMap=u0,u1
  LUT analytic : Lookup_n-D  BreakpointsForDimension1=lut_w  BreakpointsForDimension2=lut_T  Table=lut_an  ExtrapMethod=Clip  InternalRulePriority=Speed  RndMeth=Simplest
      settings: InputPortMap=u0,u1
  LUT select : MultiPortSwitch  Inputs=2  SaturateOnIntegerOverflow=off  InputSameDT=off
  MLP network : Subsystem
  Te_ref_f : Fcn  Expr=u(1)+Ts/0.05*(u(2)-u(1))
  Te_ref_f in : Mux  Inputs=2
  Te_ref_f(k-1) : UnitDelay  SampleTime=Ts  HasFrameUpgradeWarning=on
  abs Te_ref_f : Fcn  Expr=abs(u)
  abs w_u : Fcn  Expr=abs(u)
  dpsi : Fcn  Expr=((((((u(1)-u(2))>(-psi_rate*Ts))*(u(1)-u(2))+((u(1)-u(2))<=(-psi_rate*Ts))*(-psi_rate*Ts)))<(psi_rate*Ts))*((((u(1)-u(2))>(-psi_rate*Ts))*(u(1)-u(2))+((u(1)-u(2))<=(-psi_rate*Ts))*(-psi_rate*Ts)))+(((((u(1)-u(2))>(-psi_rate*Ts))*(u(1)-u(2))+((u(1)-u(2))<=(-psi_rate*Ts))*(-psi_rate*Ts)))>=(psi_rate*Ts))*(psi_rate*Ts))
  dpsi in : Mux  Inputs=2
  dpsi_rate : Fcn  Expr=u/Ts
  dpsi_rate(k-1) : UnitDelay  SampleTime=Ts  HasFrameUpgradeWarning=on
  psi_ref : Fcn  Expr=u(1)+u(2)
  psi_ref in : Mux  Inputs=2
  psi_ref(k-1) : UnitDelay  SampleTime=Ts  HasFrameUpgradeWarning=on
  psi_target : Fcn  Expr=((u(1)>0)*(psi_r_rated)+(1-(u(1)>0))*(((((((((u(2)<1.5)*(psi_r_rated)+(1-(u(2)<1.5))*(((u(2)<2.5)*(psi_fixed)+(1-(u(2)<2.5))*(((u(2)<3.5)*(u(3))+(1-(u(2)<3.5))*(u(4))))))))>(psi_min))*(((u(2)<1.5)*(psi_r_rated)+(1-(u(2)<1.5))*(((u(2)<2.5)*(psi_fixed)+(1-(u(2)<2.5))*(((u(2)<3.5)*(u(3))+(1-(u(2)<3.5))*(u(4))))))))+((((u(2)<1.5)*(psi_r_rated)+(1-(u(2)<1.5))*(((u(2)<2.5)*(psi_fixed)+(1-(u(2)<2.5))*(((u(2)<3.5)*(u(3))+(1-(u(2)<3.5))*(u(4))))))))<=(psi_min))*(psi_min)))<(psi_r_rated))*((((((u(2)<1.5)*(psi_r_rated)+(1-(u(2)<1.5))*(((u(2)<2.5)*(psi_fixed)+(1-(u(2)<2.5))*(((u(2)<3.5)*(u(3))+(1-(u(2)<3.5))*(u(4))))))))>(psi_min))*(((u(2)<1.5)*(psi_r_rated)+(1-(u(2)<1.5))*(((u(2)<2.5)*(psi_fixed)+(1-(u(2)<2.5))*(((u(2)<3.5)*(u(3))+(1-(u(2)<3.5))*(u(4))))))))+((((u(2)<1.5)*(psi_r_rated)+(1-(u(2)<1.5))*(((u(2)<2.5)*(psi_fixed)+(1-(u(2)<2.5))*(((u(2)<3.5)*(u(3))+(1-(u(2)<3.5))*(u(4))))))))<=(psi_min))*(psi_min)))+(((((((u(2)<1.5)*(psi_r_rated)+(1-(u(2)<1.5))*(((u(2)<2.5)*(psi_fixed)+(1-(u(2)<2.5))*(((u(2)<3.5)*(u(3))+(1-(u(2)<3.5))*(u(4))))))))>(psi_min))*(((u(2)<1.5)*(psi_r_rated)+(1-(u(2)<1.5))*(((u(2)<2.5)*(psi_fixed)+(1-(u(2)<2.5))*(((u(2)<3.5)*(u(3))+(1-(u(2)<3.5))*(u(4))))))))+((((u(2)<1.5)*(psi_r_rated)+(1-(u(2)<1.5))*(((u(2)<2.5)*(psi_fixed)+(1-(u(2)<2.5))*(((u(2)<3.5)*(u(3))+(1-(u(2)<3.5))*(u(4))))))))<=(psi_min))*(psi_min)))>=(psi_r_rated))*(psi_r_rated))))
  psi_target in : Mux
  trans_t : Fcn  Expr=(((((((abs(u(1))>trans_dw)+(abs(u(2)-u(3))>trans_dT))>0)*(trans_hold)+(1-(((abs(u(1))>trans_dw)+(abs(u(2)-u(3))>trans_dT))>0))*(u(4)))-Ts)>(0))*(((((abs(u(1))>trans_dw)+(abs(u(2)-u(3))>trans_dT))>0)*(trans_hold)+(1-(((abs(u(1))>trans_dw)+(abs(u(2)-u(3))>trans_dT))>0))*(u(4)))-Ts)+((((((abs(u(1))>trans_dw)+(abs(u(2)-u(3))>trans_dT))>0)*(trans_hold)+(1-(((abs(u(1))>trans_dw)+(abs(u(2)-u(3))>trans_dT))>0))*(u(4)))-Ts)<=(0))*(0))
  trans_t in : Mux
  trans_t(k-1) : UnitDelay  SampleTime=Ts  HasFrameUpgradeWarning=on
  psi_ref out : Outport
  dpsi_rate out : Outport  Port=2
  psi_ref_p out : Outport  Port=3
  trans_t_p out : Outport  Port=4
  dpsi_rate_p out : Outport  Port=5
  wires:
  e_w/1 -> trans_t in/1
  Te_ref/1 -> trans_t in/2, Te_ref_f in/2
  Te_ref_f(k-1)/1 -> trans_t in/3, Te_ref_f in/1
  trans_t(k-1)/1 -> trans_t in/4, trans_t_p out/1
  trans_t in/1 -> trans_t/1
  trans_t/1 -> trans_t(k-1)/1, psi_target in/1
  Te_ref_f in/1 -> Te_ref_f/1
  Te_ref_f/1 -> Te_ref_f(k-1)/1, abs Te_ref_f/1
  w_u/1 -> abs w_u/1
  abs w_u/1 -> LUT analytic/1, LUT ML/1, MLP network/1(w)
  abs Te_ref_f/1 -> LUT analytic/2, LUT ML/2, MLP network/2(T)
  lut_sel/1 -> LUT select/1
  LUT analytic/1 -> LUT select/2
  LUT ML/1 -> LUT select/3
  flux_sel/1 -> psi_target in/2
  LUT select/1 -> psi_target in/3
  MLP network/1(psi out) -> psi_target in/4
  psi_target in/1 -> psi_target/1
  psi_target/1 -> dpsi in/1
  psi_ref(k-1)/1 -> dpsi in/2, psi_ref in/1, psi_ref_p out/1
  dpsi in/1 -> dpsi/1
  dpsi/1 -> psi_ref in/2, dpsi_rate/1
  psi_ref in/1 -> psi_ref/1
  psi_ref/1 -> psi_ref(k-1)/1, psi_ref out/1
  dpsi_rate/1 -> dpsi_rate(k-1)/1, dpsi_rate out/1
  dpsi_rate(k-1)/1 -> dpsi_rate_p out/1

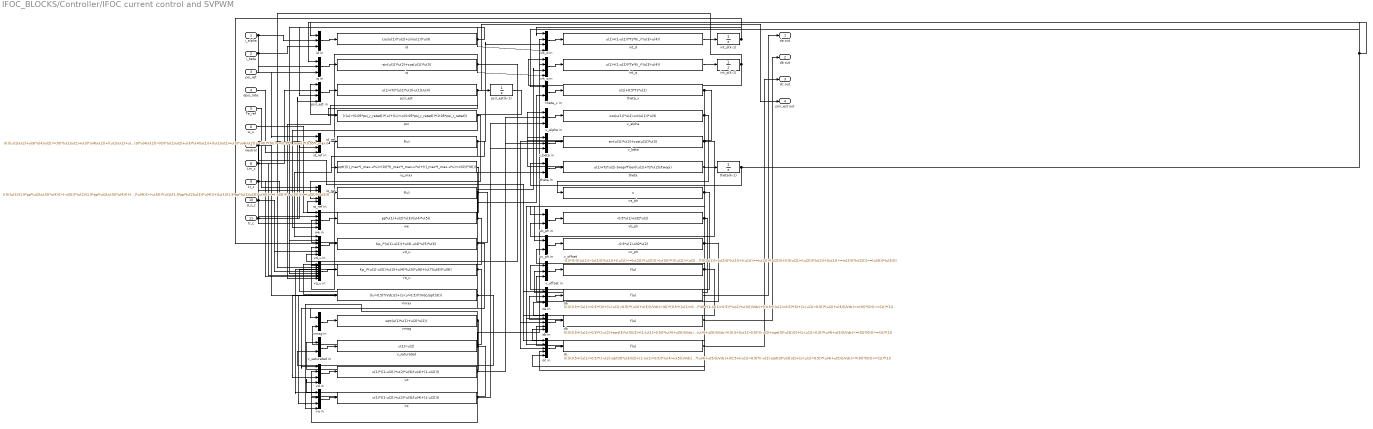
== system IFOC_BLOCKS/Controller/IFOC current control and SVPWM ==
  i_alpha : Inport
  i_beta : Inport  Port=2
  psi_ref : Inport  Port=3
  dpsi_rate : Inport  Port=4
  Te_ref : Inport  Port=5
  w_u : Inport  Port=6
  neutral : Inport  Port=7
  Lm_c : Inport  Port=8
  Lr_c : Inport  Port=9
  sLs_c : Inport  Port=10
  tr_c : Inport  Port=11
  Vmax : Fcn  Expr=((u>0.5)*(Vdc/2)+(1-(u>0.5))*(Vdc/sqrt(3)))
  da : Fcn  Expr=((((((0.5+((u(1)>0.5)*(0)+(1-(u(1)>0.5))*(u(2)+u(3)))/Vdc)>(0))*(0.5+((u(1)>0.5)*(0)+(1-(u(1)>0.5))*(u(2)+u(3)))/Vdc)+((0.5+((u(1)>0.5)*(0)+(1-(u(1)>0.5))*(u(2)+u(3)))/Vdc)<=(0))*(0)))<(1))*((((0.5+((u(1)>0.5)*(0)+(1-(u(1)>0.5))*(u(2)+u(3)))/Vdc)>(0))*(0.5+((u(1)>0.5)*(0)+(1-(u(1)>0.5))*(u(2)+u(3)))/Vdc)+((0.5+((u(1)>0.5)*(0)+(1-(u(1)>0.5))*(u(2)+u(3)))/Vdc)<=(0))*(0)))+(((((0.5+((u(1)>0.5)*(0)+(1-(u(1)>0.5))*(u(2)+u(3)))/Vdc)>(0))*(0.5+((u(1)>0.5)*(0)+(1-(u(1)>0.5))*(u(2)+u(3)))/Vdc)+((0.5+((u(1)>0.5)*(0)+(1-(u(1)>0.5))*(u(2)+u(3)))/Vdc)<=(0))*(0)))>=(1))*(1))
  da in : Mux  Inputs=3
  db : Fcn  Expr=((((((0.5+((u(1)>0.5)*((-u(2)+sqrt(3)*u(3))/2)+(1-(u(1)>0.5))*(u(4)+u(5)))/Vdc)>(0))*(0.5+((u(1)>0.5)*((-u(2)+sqrt(3)*u(3))/2)+(1-(u(1)>0.5))*(u(4)+u(5)))/Vdc)+((0.5+((u(1)>0.5)*((-u(2)+sqrt(3)*u(3))/2)+(1-(u(1)>0.5))*(u(4)+u(5)))/Vdc)<=(0))*(0)))<(1))*((((0.5+((u(1)>0.5)*((-u(2)+sqrt(3)*u(3))/2)+(1-(u(1)>0.5))*(u(4)+u(5)))/Vdc)>(0))*(0.5+((u(1)>0.5)*((-u(2)+sqrt(3)*u(3))/2)+(1-(u(1)>0.5))*(u(4)+u(5)))/Vdc)+((0.5+((u(1)>0.5)*((-u(2)+sqrt(3)*u(3))/2)+(1-(u(1)>0.5))*(u(4)+u(5)))/Vdc)<=(0))*(0)))+(((((0.5+((u(1)>0.5)*((-u(2)+sqrt(3)*u(3))/2)+(1-(u(1)>0.5))*(u(4)+u(5)))/Vdc)>(0))*(0.5+((u(1)>0.5)*((-u(2)+sqrt(3)*u(3))/2)+(1-(u(1)>0.5))*(u(4)+u(5)))/Vdc)+((0.5+((u(1)>0.5)*((-u(2)+sqrt(3)*u(3))/2)+(1-(u(1)>0.5))*(u(4)+u(5)))/Vdc)<=(0))*(0)))>=(1))*(1))
  db in : Mux  Inputs=5
  dc : Fcn  Expr=((((((0.5+((u(1)>0.5)*((-u(2)-sqrt(3)*u(3))/2)+(1-(u(1)>0.5))*(u(4)+u(5)))/Vdc)>(0))*(0.5+((u(1)>0.5)*((-u(2)-sqrt(3)*u(3))/2)+(1-(u(1)>0.5))*(u(4)+u(5)))/Vdc)+((0.5+((u(1)>0.5)*((-u(2)-sqrt(3)*u(3))/2)+(1-(u(1)>0.5))*(u(4)+u(5)))/Vdc)<=(0))*(0)))<(1))*((((0.5+((u(1)>0.5)*((-u(2)-sqrt(3)*u(3))/2)+(1-(u(1)>0.5))*(u(4)+u(5)))/Vdc)>(0))*(0.5+((u(1)>0.5)*((-u(2)-sqrt(3)*u(3))/2)+(1-(u(1)>0.5))*(u(4)+u(5)))/Vdc)+((0.5+((u(1)>0.5)*((-u(2)-sqrt(3)*u(3))/2)+(1-(u(1)>0.5))*(u(4)+u(5)))/Vdc)<=(0))*(0)))+(((((0.5+((u(1)>0.5)*((-u(2)-sqrt(3)*u(3))/2)+(1-(u(1)>0.5))*(u(4)+u(5)))/Vdc)>(0))*(0.5+((u(1)>0.5)*((-u(2)-sqrt(3)*u(3))/2)+(1-(u(1)>0.5))*(u(4)+u(5)))/Vdc)+((0.5+((u(1)>0.5)*((-u(2)-sqrt(3)*u(3))/2)+(1-(u(1)>0.5))*(u(4)+u(5)))/Vdc)<=(0))*(0)))>=(1))*(1))
  dc in : Mux  Inputs=5
  id : Fcn  Expr=cos(u(1))*u(2)+sin(u(1))*u(3)
  id in : Mux  Inputs=3
  id_ref : Fcn  Expr=((((((u(1)/u(2)+u(3)*u(4)/u(2))>(0))*(u(1)/u(2)+u(3)*u(4)/u(2))+((u(1)/u(2)+u(3)*u(4)/u(2))<=(0))*(0)))<(0.95*I_max))*((((u(1)/u(2)+u(3)*u(4)/u(2))>(0))*(u(1)/u(2)+u(3)*u(4)/u(2))+((u(1)/u(2)+u(3)*u(4)/u(2))<=(0))*(0)))+(((((u(1)/u(2)+u(3)*u(4)/u(2))>(0))*(u(1)/u(2)+u(3)*u(4)/u(2))+((u(1)/u(2)+u(3)*u(4)/u(2))<=(0))*(0)))>=(0.95*I_max))*(0.95*I_max))
  id_ref in : Mux
  int_d : Fcn  Expr=u(1)+(1-u(2))*Ts*Ki_i*(u(3)-u(4))
  int_d in : Mux
  int_d(k-1) : UnitDelay  SampleTime=Ts  HasFrameUpgradeWarning=on
  int_q : Fcn  Expr=u(1)+(1-u(2))*Ts*Ki_i*(u(3)-u(4))
  int_q in : Mux
  int_q(k-1) : UnitDelay  SampleTime=Ts  HasFrameUpgradeWarning=on
  iq : Fcn  Expr=-sin(u(1))*u(2)+cos(u(1))*u(3)
  iq in : Mux  Inputs=3
  iq_max : Fcn  Expr=sqrt((((I_max*I_max-u*u)>(0))*(I_max*I_max-u*u)+((I_max*I_max-u*u)<=(0))*(0)))
  iq_ref : Fcn  Expr=((((((u(1)/(1.5*pp*(u(2)/u(3))*u(4)))>(-u(5)))*(u(1)/(1.5*pp*(u(2)/u(3))*u(4)))+((u(1)/(1.5*pp*(u(2)/u(3))*u(4)))<=(-u(5)))*(-u(5))))<(u(5)))*((((u(1)/(1.5*pp*(u(2)/u(3))*u(4)))>(-u(5)))*(u(1)/(1.5*pp*(u(2)/u(3))*u(4)))+((u(1)/(1.5*pp*(u(2)/u(3))*u(4)))<=(-u(5)))*(-u(5))))+(((((u(1)/(1.5*pp*(u(2)/u(3))*u(4)))>(-u(5)))*(u(1)/(1.5*pp*(u(2)/u(3))*u(4)))+((u(1)/(1.5*pp*(u(2)/u(3))*u(4)))<=(-u(5)))*(-u(5))))>=(u(5)))*(u(5)))
  iq_ref in : Mux  Inputs=5
  psir_est : Fcn  Expr=u(1)+Ts*(u(2)*u(3)-u(1))/u(4)
  psir_est in : Mux
  psir_est(k-1) : UnitDelay  SampleTime=Ts  HasFrameUpgradeWarning=on
  psr : Fcn  Expr=(((u)>(0.05*psi_r_rated))*(u)+((u)<=(0.05*psi_r_rated))*(0.05*psi_r_rated))
  theta : Fcn  Expr=u(1)+Ts*u(2)-twopi*floor((u(1)+Ts*u(2))/twopi)
  theta in : Mux  Inputs=2
  theta(k-1) : UnitDelay  SampleTime=Ts  HasFrameUpgradeWarning=on
  theta_v : Fcn  Expr=u(1)+0.5*Ts*u(2)
  theta_v in : Mux  Inputs=2
  v_alpha : Fcn  Expr=cos(u(1))*u(2)-sin(u(1))*u(3)
  v_alpha in : Mux  Inputs=3
  v_beta : Fcn  Expr=sin(u(1))*u(2)+cos(u(1))*u(3)
  v_beta in : Mux  Inputs=3
  v_offset : Fcn  Expr=-0.5*(((((((u(1))>(u(2)))*(u(1))+((u(1))<=(u(2)))*(u(2))))>(u(3)))*((((u(1))>(u(2)))*(u(1))+((u(1))<=(u(2)))*(u(2))))+(((((u(1))>(u(2)))*(u(1))+((u(1))<=(u(2)))*(u(2))))<=(u(3)))*(u(3)))+((((((u(1))<(u(2)))*(u(1))+((u(1))>=(u(2)))*(u(2))))<(u(3)))*((((u(1))<(u(2)))*(u(1))+((u(1))>=(u(2)))*(u(2))))+(((((u(1))<(u(2)))*(u(1))+((u(1))>=(u(2)))*(u(2))))>=(u(3)))*(u(3))))
  v_offset in : Mux  Inputs=3
  v_saturated : Fcn  Expr=u(1)>u(2)
  v_saturated in : Mux  Inputs=2
  va_ph : Fcn  Expr=u
  vb_ph : Fcn  Expr=-0.5*u(1)+s32*u(2)
  vb_ph in : Mux  Inputs=2
  vc_ph : Fcn  Expr=-0.5*u(1)-s32*u(2)
  vc_ph in : Mux  Inputs=2
  vd : Fcn  Expr=u(1)*((1-u(2))+u(2)*u(3)/(u(4)+(1-u(2))))
  vd in : Mux
  vd_u : Fcn  Expr=Kp_i*(u(1)-u(2))+u(3)-u(4)*u(5)*u(6)
  vd_u in : Mux  Inputs=6
  vmag : Fcn  Expr=sqrt(u(1)*u(1)+u(2)*u(2))
  vmag in : Mux  Inputs=2
  vq : Fcn  Expr=u(1)*((1-u(2))+u(2)*u(3)/(u(4)+(1-u(2))))
  vq in : Mux
  vq_u : Fcn  Expr=Kp_i*(u(1)-u(2))+u(3)+u(4)*(u(5)*u(6)+(u(7)/u(8))*u(9))
  vq_u in : Mux  Inputs=9
  we : Fcn  Expr=pp*u(1)+u(2)*u(3)/(u(4)*u(5))
  we in : Mux  Inputs=5
  da out : Outport
  db out : Outport  Port=2
  dc out : Outport  Port=3
  psir_est out : Outport  Port=4
  wires:
  theta(k-1)/1 -> id in/1, iq in/1, theta_v in/1, theta in/1
  i_alpha/1 -> id in/2, iq in/2
  i_beta/1 -> id in/3, iq in/3
  id in/1 -> id/1
  iq in/1 -> iq/1
  psir_est(k-1)/1 -> psir_est in/1
  Lm_c/1 -> psir_est in/2, id_ref in/2, iq_ref in/2, we in/2, vq_u in/7
  id/1 -> psir_est in/3, vd_u in/2, vq_u in/6, int_d in/4
  tr_c/1 -> psir_est in/4, id_ref in/3, we in/4
  psir_est in/1 -> psir_est/1
  psir_est/1 -> psir_est(k-1)/1, psr/1, vq_u in/9, psir_est out/1
  psi_ref/1 -> id_ref in/1
  dpsi_rate/1 -> id_ref in/4
  id_ref in/1 -> id_ref/1
  id_ref/1 -> iq_max/1, vd_u in/1, int_d in/3
  Te_ref/1 -> iq_ref in/1
  Lr_c/1 -> iq_ref in/3, vq_u in/8
  psr/1 -> iq_ref in/4, we in/5
  iq_max/1 -> iq_ref in/5
  iq_ref in/1 -> iq_ref/1
  w_u/1 -> we in/1
  iq_ref/1 -> we in/3, vq_u in/1, int_q in/3
  we in/1 -> we/1
  int_d(k-1)/1 -> vd_u in/3, int_d in/1
  we/1 -> vd_u in/4, vq_u in/4, theta_v in/2, theta in/2
  sLs_c/1 -> vd_u in/5, vq_u in/5
  iq/1 -> vd_u in/6, vq_u in/2, int_q in/4
  vd_u in/1 -> vd_u/1
  int_q(k-1)/1 -> vq_u in/3, int_q in/1
  vq_u in/1 -> vq_u/1
  neutral/1 -> Vmax/1, da in/1, db in/1, dc in/1
  vd_u/1 -> vmag in/1, vd in/1
  vq_u/1 -> vmag in/2, vq in/1
  vmag in/1 -> vmag/1
  vmag/1 -> v_saturated in/1, vd in/4, vq in/4
  Vmax/1 -> v_saturated in/2, vd in/3, vq in/3
  v_saturated in/1 -> v_saturated/1
  v_saturated/1 -> vd in/2, vq in/2, int_d in/2, int_q in/2
  vd in/1 -> vd/1
  vq in/1 -> vq/1
  int_d in/1 -> int_d/1
  int_d/1 -> int_d(k-1)/1
  int_q in/1 -> int_q/1
  int_q/1 -> int_q(k-1)/1
  theta_v in/1 -> theta_v/1
  theta_v/1 -> v_alpha in/1, v_beta in/1
  vd/1 -> v_alpha in/2, v_beta in/2
  vq/1 -> v_alpha in/3, v_beta in/3
  v_alpha in/1 -> v_alpha/1
  v_beta in/1 -> v_beta/1
  theta in/1 -> theta/1
  theta/1 -> theta(k-1)/1
  v_alpha/1 -> va_ph/1, vb_ph in/1, vc_ph in/1, db in/2, dc in/2
  v_beta/1 -> vb_ph in/2, vc_ph in/2, db in/3, dc in/3
  vb_ph in/1 -> vb_ph/1
  vc_ph in/1 -> vc_ph/1
  va_ph/1 -> v_offset in/1, da in/2
  vb_ph/1 -> v_offset in/2, db in/4
  vc_ph/1 -> v_offset in/3, dc in/4
  v_offset in/1 -> v_offset/1
  v_offset/1 -> da in/3, db in/5, dc in/5
  da in/1 -> da/1
  db in/1 -> db/1
  dc in/1 -> dc/1
  da/1 -> da out/1
  db/1 -> db out/1
  dc/1 -> dc out/1
